simulink model "jumeau_banc_rw"  (R2025b)
settings: Solver=ode23t  StartTime=0.0  StopTime=20  MaxStep=1e-3  RelTol=1e-4
PostLoadFcn:
  | d = fileparts(get_param('jumeau_banc_rw', 'FileName')); addpath(fullfile(d, 'geometrie'), fullfile(d, 'liaison'), fullfile(d, 'pilotage')); clear d
StartFcn:
  | % Jumeau Webots : au lancement, MATLAB envoie les paramètres du Model Workspace à Webots, qui remet le banc en
  | % position de départ, puis ouvre la liaison de télémétrie et la liaison de commande (liaison/pont_banc.m).
  | if strcmp(get_param('jumeau_banc_rw/Procédé', 'LabelModeActiveChoice'), 'Webots')
  |     pont_banc('ouvrir', getVariable(get_param('jumeau_banc_rw', 'ModelWorkspace'), 'config_jumeau'));
  | end
  | pilotage_banc('depart');   % interface de pilotage : nouveau lancement
StopFcn:
  | pont_banc('fermer');
  | pilotage_banc('fin');
model workspace (MATLAB code in the model file):
  | %% Jumeau numérique du banc de stabilisation à 4 roues de réaction (version 3) : paramètres
  | % Ce code est enregistré dans le modèle (Model Explorer > jumeau_banc_rw > Model Workspace).
  | % Origine : (CAO) CAO du banc version 3, (M) mesuré sur le matériel, (F) fiche technique, (Fw) firmware,
  | % (H) hypothèse à mesurer sur le banc. Masses et inerties des pièces : dans chaque bloc de pièce.
  | 
  | %% Montage de l'essai
  | pivot_mm = 25;              % position du pivot de tangage sur le corps : 25, 24, 16, 8, 0, -8 mm (25 : banc équilibré, rangée +24 et paliers remontés de 1 mm)
  | blocage_roulis = 0;         % goupille de blocage : 1 = axe bloqué à 0°, 0 = axe libre
  | blocage_tangage = 0;
  | angle0_roulis_deg = 2;      % position de départ (mise à 0 si l'axe est bloqué)
  | angle0_tangage_deg = -1;
  | g = 9.81;                   % m/s²
  | 
  | %% Pupitre : pilotage manuel des 4 ESC
  | essai_t = 1;                % s, instant de l'échelon d'essai ajouté aux curseurs
  | essai_echelon_us = [0 0 0 0];   % µs, échelon d'essai sur chaque ESC (0 : aucun)
  | 
  | %% Alimentation des ESC
  | V_alim = 12;                % V, alimentation de labo (H : tension réglée)
  | 
  | %% ESC Brushless 30A bidirectionnels (x4)
  | f_trame_esc = 50;           % Hz, une impulsion toutes les 20 ms (Fw : LEDC 50 Hz)
  | imp_neutre = 1500;          % µs, neutre (testé sur le banc)
  | imp_min = 1000;             % µs (Fw)
  | imp_max = 2000;             % µs (Fw)
  | zone_morte_us = 0;          % µs autour du neutre (H)
  | tau_esc = 2e-3;             % s, temps de réponse de l'ESC (H)
  | armement_actif = 1;         % 1 : l'ESC ne pilote le moteur qu'après t_armement au neutre
  | t_armement = 1;             % s (H)
  | fenetre_armement_us = 25;   % µs, écart au neutre accepté pendant l'armement (H)
  | sens_moteurs = [1 1 1 1];   % +1 : au-dessus du neutre, la roue tourne dans le sens +axe (vers l'extérieur) (H : ordre des phases)
  | 
  | %% Moteurs A2212 1400 KV (x4), modèle équivalent continu
  | KV = 1400;                  % tr/min/V (F)
  | Ke = 60/(2*pi*KV);          % V.s/rad
  | Kt = Ke;                    % N.m/A
  | R_moteur = 0.08;            % ohm (H)
  | L_moteur = 30e-6;           % H (H)
  | f_roue = 5e-6;              % N.m.s/rad, frottement visqueux des roulements du moteur (H)
  | 
  | %% Cardan
  | butee_deg = 20;             % débattement de chaque axe (CAO)
  | k_butee = 20;               % N.m/rad, contact goupille-lumière (H)
  | c_butee = 0.2;              % N.m.s/rad (H)
  | b_cardan = 1e-4;            % N.m.s/rad, frottement des roulements 625 (H)
  | k_cables = 0;               % N.m/rad, raideur des deux câbles vers la table (H)
  | 
  | %% BNO055 (mode fusion)
  | T_bno = 0.01;               % s, données de fusion à 100 Hz (F)
  | bruit_bno = 1;              % 1 : bruit de mesure, 0 : capteur parfait
  | sigma_angle_deg = 0.05;     % ° (H)
  | sigma_gyro_dps = 0.1;       % °/s (H)
  | sigma_acc = 0.02;           % m/s² (H)
  | R_montage_bno = eye(3);     % axes du capteur dans le repère du dispositif : eye(3) = remappage AXIS_MAP réglé
  |                             % (la carte est tournée de 90° dans la CAO)
  | 
  | %% Capteurs de vitesse TCRT5000 (x4) : un front à chaque rayon du disque
  | n_rayons = 4;               % rayons du disque vus par tour (CAO : disque d'origine)
  | T_tcrt = 1e-3;              % s, pas de calcul du capteur (les fronts sont datés par interpolation, comme un chronomètre en µs)
  | t_arret_tcrt = 0.2;         % s sans front : la vitesse mesurée retombe à 0 (Fw, à fixer)
  | 
  | %% Pont vers le jumeau Webots (et, plus tard, vers l'ESP32 du banc réel)
  | T_pont = 0.01;              % s, une trame de commande et une trame de télémétrie toutes les 10 ms
  | 
  | %% Essai : maintien au départ et perturbation
  | t_lacher = 2;                % s, le dispositif est tenu à la main à sa position de départ jusqu'à cet instant (0 : libre dès le départ)
  | k_main = 5;                  % N.m/rad, raideur de la main qui tient le dispositif
  | c_main = 0.3;                % N.m.s/rad, son amortissement
  | perturbation_t = 7;          % s, instant de la poussée d'essai
  | perturbation_duree = 0.2;    % s
  | perturbation_couple = [0.02 0.02];   % N.m, couple de la poussée sur [roulis tangage], programmée (0 : aucune ; l'interface de pilotage en ajoute)
  | 
  | %% Grandeurs dérivées
  | assert(any(pivot_mm == [25 24 16 8 0 -8]), 'pivot_mm : 25, 24, 16, 8, 0, -8');
  | q0_deg = [angle0_roulis_deg angle0_tangage_deg] .* ([blocage_roulis blocage_tangage] == 0);
  | config_jumeau = [pivot_mm; blocage_roulis; blocage_tangage; q0_deg(:); V_alim; f_trame_esc; imp_neutre; imp_min; imp_max; ...
  |     zone_morte_us; tau_esc; armement_actif; t_armement; fenetre_armement_us; sens_moteurs(:); Ke; Kt; R_moteur; L_moteur; ...
  |     f_roue; butee_deg; k_butee; c_butee; b_cardan; k_cables; g; T_bno; bruit_bno; sigma_angle_deg; sigma_gyro_dps; ...
  |     sigma_acc; n_rayons; t_arret_tcrt; T_tcrt; R_montage_bno(:); T_pont; t_lacher; k_main; c_main];   % 51 valeurs envoyées au jumeau Webots au lancement
  | 
  | %% Commande bas niveau : une boucle de vitesse par roue, avec observateur CFO (méthode du TP2, ramenée à la vitesse)
  | J_roue = 1.562e-4;          % kg.m², inertie d'une roue autour de son axe : disque, vis, cloche du moteur (CAO)
  | T_cbn = 1/f_trame_esc;      % s, période de calcul de la commande : celle des ESC, qui ne lisent qu'une impulsion toutes les 20 ms
  | wc_roue = [10 10 10 10];    % rad/s, rapidité du suivi de vitesse de chaque roue (pôle de l'erreur en -wc)
  | wo_roue = [5 5 5 5];        % rad/s, rapidité du CFO de chaque roue (pôles en -wo et -4 wo) ; au-delà de 10, il devient instable à 20 ms
  | imp_cmd_min = 1375;         % µs, limites des impulsions commandées : vitesse conseillée des disques, 3 900 tr/min
  | imp_cmd_max = 1625;         % µs
  | w_aveugle = 45;             % rad/s, en dessous (vitesse du modèle), le TCRT5000 voit mal la roue : le CFO ne se corrige plus sur la mesure
  | 
  | %% Consigne d'essai des roues : ajoutée à la consigne qui vient de la conversion (0 tant qu'elle est vide)
  | essai_roue_t1 = 2;                  % s, départ vers le premier palier
  | essai_roue_vitesse1 = [0 0 0 0];  % rad/s, premier palier de chaque roue (0 : la roue reste à l'arrêt)
  | essai_roue_t2 = 6;                  % s, départ vers le second palier
  | essai_roue_vitesse2 = [0 0 0 0];    % rad/s, second palier de chaque roue
  | essai_roue_acc = 300;               % rad/s², pente des rampes entre les paliers
  | 
  | %% Commande bas niveau : grandeurs calculées
  | % modèle local d'une roue : d(omega)/dt = -a1 omega + a0 V + d
  | a0_roue = Kt/(R_moteur*J_roue) * [1 1 1 1];                % rad/s² par volt
  | a1_roue = (Kt*Ke/R_moteur + f_roue)/J_roue * [1 1 1 1];    % 1/s
  | K_roue = wc_roue - a1_roue;                                % retour d'état : erreur en -(a1 + K) = -wc
  | l1_roue = 5*wo_roue;                                       % CFO
  | lambda_roue = 4/5*wo_roue;
  | 
  | %% Référence : angles demandés au dispositif, en polynômes de degré 5 entre deux paliers
  | ref_t = [2 12];              % s, instant de départ vers chaque palier
  | ref_roulis_deg = [0 5];      % °, roulis demandé à chaque palier
  | ref_tangage_deg = [0 0];     % °, tangage demandé à chaque palier
  | ref_duree = 1.5;             % s, durée du passage d'un palier au suivant
  | 
  | %% Commande haut niveau : une boucle par axe [roulis tangage], placement de pôles basé sur l'observateur CFO (TP2)
  | T_chn = T_cbn;               % s, période de calcul : celle de la commande bas niveau et des ESC
  | t_depart = t_lacher;         % s, mise en marche de la commande : au moment où la main lâche le dispositif
  | wc_axe = [4 4];              % rad/s, rapidité du suivi d'angle de chaque axe
  | xi_axe = [1 1];              % amortissement
  | wo_axe = [3 3];              % rad/s, rapidité du CFO de chaque axe (pôles en -wo et -4 wo, double) ; au-delà de 4, le couple s'agite
  | desat_active = 0;            % 1 : la référence est décalée pour ramener les roues vers leur vitesse de repos
  | T_desat = 5;                 % s, constante de temps de ce retour
  | desat_max_deg = 15;          % °, décalage maximal de la référence
  | 
  | %% Conversion : couples des deux axes vers les 4 roues
  | w_repos = 200;               % rad/s, vitesse de repos des 4 roues : elles tournent toujours, le TCRT5000 les voit toujours
  | t_roues = t_armement + 0.2;  % s, mise en rotation des roues, une fois les ESC armés
  | acc_roue_max = 300;          % rad/s², accélération maximale demandée à une roue
  | w_roue_min = 60;             % rad/s, vitesses limites demandées à une roue
  | w_roue_max = 400;            % rad/s (disques : 3 900 tr/min conseillés, soit 408 rad/s)
  | 
  | %% Masses et inerties utilisées par la commande (CAO du banc version 3)
  | m_disp = 1.2615;             % kg, dispositif et ses 4 roues
  | zG_disp = 24.977e-3;         % m, hauteur de son centre de masse sur le corps (le pivot est à pivot_mm)
  | Ixx_disp_24 = 8.2684e-3;     % kg.m², inertie du dispositif autour du roulis, pivot à +24 mm
  | Iyy_disp_24 = 8.2786e-3;     % kg.m², autour du tangage, pivot à +24 mm
  | m_croix = 0.0755;            % kg, croisillon et paliers (ne tournent qu'en roulis)
  | zG_croix = 0.257e-3;         % m, hauteur de leur centre de masse au-dessus de l'axe de roulis
  | Ixx_croix = 2.073e-4;        % kg.m²
  | 
  | %% Commande haut niveau et conversion : grandeurs calculées
  | % modèle local d'un axe : d²(theta)/dt² = -a1 d(theta)/dt + a0 C + d, avec C le couple demandé aux roues
  | hz = zG_disp - pivot_mm/1000;                                    % m, centre de masse du dispositif au-dessus du pivot
  | I_axe = [Ixx_disp_24 + Ixx_croix, Iyy_disp_24] + m_disp*(hz^2 - (zG_disp - 0.024)^2) - 2*J_roue;   % kg.m²
  | mgh_axe = g*[m_disp*hz + m_croix*zG_croix, m_disp*hz];           % N.m/rad, couple de pesanteur par radian d'inclinaison
  | a0_axe = 1./I_axe;                                               % rad/s² par N.m
  | a1_axe = b_cardan./I_axe;                                        % 1/s
  | k1_axe = wc_axe.^2;                                              % retour d'état : s² + 2 xi wc s + wc²
  | k2_axe = 2*xi_axe.*wc_axe - a1_axe;
  | l1_axe = 9*wo_axe;                                               % CFO du TP2
  | l2_axe = 12*wo_axe.^2;
  | lambda_axe = 4/3*wo_axe;
  | C_max = 2*J_roue*cosd(45)*acc_roue_max;                          % N.m, couple maximal demandé sur un axe
  | k_desat = desat_active.*sign(mgh_axe + (mgh_axe == 0))./(max(abs(mgh_axe), 1e-3)*T_desat);            % rad par N.m.s
  | sx_roues = [1 -1 -1 1];                                          % signe de cos(45°, 135°, 225°, 315°) : part de chaque roue sur le roulis
  | sy_roues = [1 1 -1 -1];                                          % signe de sin : part sur le tangage
  | M_conv = -[sx_roues(:) sy_roues(:)]/(4*J_roue*cosd(45));         % accélération des 4 roues pour un couple [roulis; tangage]
  | 
  | %% Perception : des mesures à l'état du banc
  | T_perception = T_bno;        % s, période de calcul : celle du BNO055
  | tau_desequilibre = 2;        % s, constante de temps du filtre du couple extérieur et du déséquilibre
  | 
  | %% Pilotage par l'interface (pilotage/pilote_banc.m)
  | manche_max_deg = 15;         % °, limite de sécurité de l'inclinaison demandée par le manche (l'interface règle l'amplitude)
  | w_manche = 3;                % rad/s, rapidité avec laquelle la référence rejoint le manche (second ordre critique)
  | T_affichage = 0.1;           % s, rafraîchissement de l'interface
undefined symbols (not defined in the file): DiscIntNeverNeededParam, X, Y, Z
libraries: sm_lib x256, nesl_utility x24, simulink x7
(part 2 of 8)

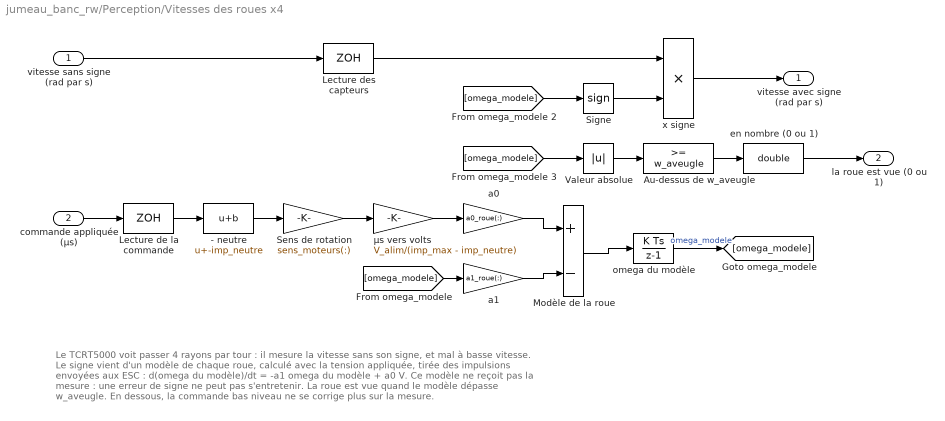
== system jumeau_banc_rw/Perception/Vitesses des roues x4 ==
  note: Le TCRT5000 voit passer 4 rayons par tour : il mesure la vitesse sans son signe, et mal à basse vitesse.
      | Le signe vient d'un modèle de chaque roue, calculé avec la tension appliquée, tirée des impulsions envoyées aux ESC :
      | d(omega du modèle)/dt = -a1 omega du modèle + a0 V. Ce modèle ne reçoit pas la mesure : une erreur de signe ne peut pas s'entretenir.
      | La roue est vue quand le modèle dépasse w_aveugle. En dessous, la commande bas niveau ne se corrige plus sur la mesure.
  vitesse sans signe (rad par s) : Inport
  commande appliquée (µs) : Inport  Port=2
  - neutre : Bias  Bias=-imp_neutre  SaturateOnIntegerOverflow=off
  Au-dessus de w_aveugle : simulink/Logic and Bit Operations/Compare To Constant  relop=>=  const=w_aveugle  OutDataTypeStr=boolean
  Lecture de la commande : ZeroOrderHold  SampleTime=T_perception
  Lecture des capteurs : ZeroOrderHold  SampleTime=T_perception
  Modèle de la roue : Sum  Inputs=+-
  Sens de rotation : Gain  Gain=sens_moteurs(:)
  Signe : Signum
  Valeur absolue : Abs  SaturateOnIntegerOverflow=off
  a0 : Gain  Gain=a0_roue(:)
  a1 : Gain  Gain=a1_roue(:)
  en nombre (0 ou 1) : DataTypeConversion  OutDataTypeStr=double  SaturateOnIntegerOverflow=off  RndMeth=Floor
  omega du modèle : DiscreteIntegrator  gainval=1  SampleTime=T_perception  ICPrevOutput=DiscIntNeverNeededParam  ICPrevScaledInput=DiscIntNeverNeededParam
  x signe : Product
  µs vers volts : Gain  Gain=V_alim/(imp_max - imp_neutre)
  vitesse avec signe (rad par s) : Outport
  la roue est vue (0 ou 1) : Outport  Port=2
  wires:
  vitesse sans signe (rad par s)/1 -> Lecture des capteurs/1
  Lecture des capteurs/1 -> x signe/1
  commande appliquée (µs)/1 -> Lecture de la commande/1
  Lecture de la commande/1 -> - neutre/1
  - neutre/1 -> Sens de rotation/1
  Sens de rotation/1 -> µs vers volts/1
  µs vers volts/1 -> a0/1
  a0/1 -> Modèle de la roue/1
  [omega_modele] -> a1/1
  a1/1 -> Modèle de la roue/2
  Modèle de la roue/1 -> omega du modèle/1
  omega du modèle/1 -> [omega_modele]  "omega_modele"
  [omega_modele] -> Signe/1
  Signe/1 -> x signe/2
  x signe/1 -> vitesse avec signe (rad par s)/1
  [omega_modele] -> Valeur absolue/1
  Valeur absolue/1 -> Au-dessus de w_aveugle/1
  Au-dessus de w_aveugle/1 -> en nombre (0 ou 1)/1
  en nombre (0 ou 1)/1 -> la roue est vue (0 ou 1)/1

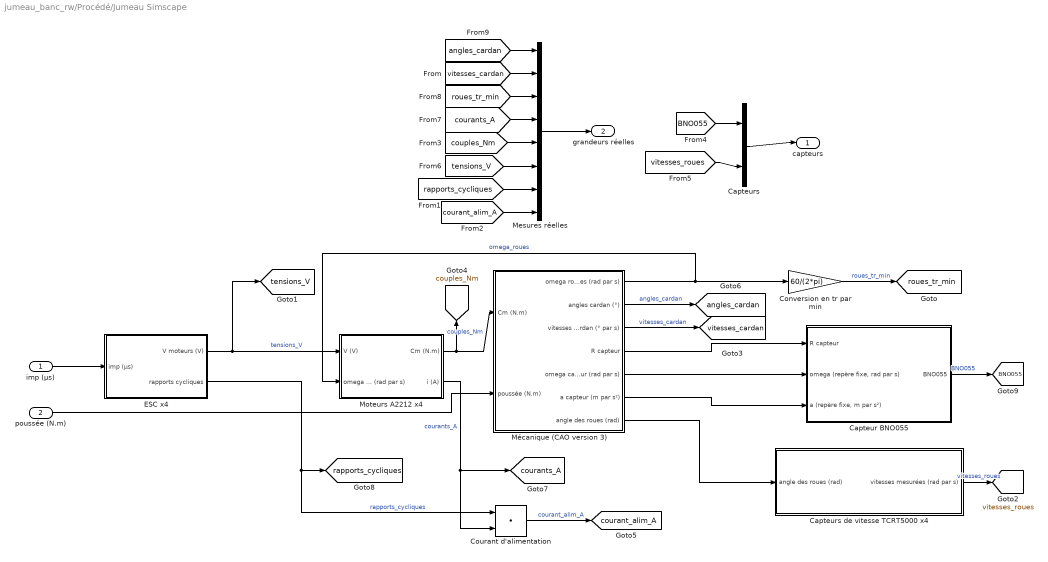
== system jumeau_banc_rw/Procédé/Jumeau Simscape ==
  imp (µs) : Inport
  poussée (N.m) : Inport  Port=2
  Capteur BNO055 : Subsystem
  Capteurs : BusCreator  Inputs=2
  Capteurs de vitesse TCRT5000 x4 : Subsystem
  Conversion en tr par min : Gain  Gain=60/(2*pi)
  Courant d'alimentation : DotProduct  OutDataTypeStr=Inherit: Inherit via internal rule
  ESC x4 : Subsystem
  Mesures réelles : BusCreator  Description=Grandeurs du banc réel, sans bruit : ce que le BNO055 et l'ESP32 ne voient pas.  Inputs=8
  Moteurs A2212 x4 : Subsystem
  Mécanique (CAO version 3) : Subsystem
  capteurs : Outport
  grandeurs réelles : Outport  Port=2
  tag scope: BNO055=global, angles_cardan=global, couples_Nm=global, courant_alim_A=global, courants_A=global, rapports_cycliques=global, roues_tr_min=global, tensions_V=global, vitesses_cardan=global, vitesses_roues=global
  wires:
  imp (µs)/1 -> ESC x4/1(imp (µs))
  ESC x4/1(V moteurs (V)) -> [tensions_V], Moteurs A2212 x4/1(V (V))  "tensions_V"
  Moteurs A2212 x4/1(Cm (N.m)) -> Mécanique (CAO version 3)/1(Cm (N.m)), [couples_Nm]  "couples_Nm"
  Mécanique (CAO version 3)/1(omega roues (rad par s)) -> Conversion en tr par min/1, Moteurs A2212 x4/2(omega roues (rad par s))  "omega_roues"
  Mécanique (CAO version 3)/4(R capteur) -> Capteur BNO055/1(R capteur)
  Mécanique (CAO version 3)/5(omega capteur (rad par s)) -> Capteur BNO055/2("omega (repère fixe, rad par s)")
  Mécanique (CAO version 3)/6(a capteur (m par s²)) -> Capteur BNO055/3("a (repère fixe, m par s²)")
  Mécanique (CAO version 3)/7(angle des roues (rad)) -> Capteurs de vitesse TCRT5000 x4/1(angle des roues (rad))
  Capteurs/1 -> capteurs/1
  ESC x4/2(rapports cycliques) -> [rapports_cycliques], Courant d'alimentation/1  "rapports_cycliques"
  Moteurs A2212 x4/2(i (A)) -> Courant d'alimentation/2, [courants_A]  "courants_A"
  Mécanique (CAO version 3)/2(angles cardan (°)) -> [angles_cardan]  "angles_cardan"
  Mécanique (CAO version 3)/3(vitesses cardan (° par s)) -> [vitesses_cardan]  "vitesses_cardan"
  Mesures réelles/1 -> grandeurs réelles/1
  [angles_cardan] -> Mesures réelles/1
  [vitesses_cardan] -> Mesures réelles/2
  Conversion en tr par min/1 -> [roues_tr_min]  "roues_tr_min"
  [roues_tr_min] -> Mesures réelles/3
  [courants_A] -> Mesures réelles/4
  [couples_Nm] -> Mesures réelles/5
  [tensions_V] -> Mesures réelles/6
  [rapports_cycliques] -> Mesures réelles/7
  [courant_alim_A] -> Mesures réelles/8
  Courant d'alimentation/1 -> [courant_alim_A]  "courant_alim_A"
  [BNO055] -> Capteurs/1
  [vitesses_roues] -> Capteurs/2
  Capteur BNO055/1(BNO055) -> [BNO055]  "BNO055"
  Capteurs de vitesse TCRT5000 x4/1(vitesses mesurées (rad par s)) -> [vitesses_roues]  "vitesses_roues"
  poussée (N.m)/1 -> Mécanique (CAO version 3)/2(poussée (N.m))

== system jumeau_banc_rw/Procédé/Jumeau Webots ==
  note: Jumeau Webots : le même banc, calculé par Webots (physique ODE, vue 3D). Lancer Webots avant la simulation :
      | ouvrir webots/worlds/banc_stabilisation.wbt, puis lancer ce modèle. Webots avance au rythme de Simulink, 10 ms par trame.
      | Liaison locale (liaison/pont_banc.m) : télémétrie reçue sur le port 5005, commande envoyée sur le port 5006 ; ce sont les trames
      | du banc réel : il suffira de remplacer Webots par l'ESP32.
      | Au lancement, les paramètres du Model Workspace (ESC, moteurs, cardan, capteurs, montage de l'essai) sont envoyés à Webots
      | (port 5007, rappel StartFcn du modèle) : MATLAB reste la seule source des réglages. Webots remet alors le banc en position de départ.
  note: Trame de commande du jumeau : les 13 octets de l'ESP32, plus la poussée d'essai (8 octets) avant la somme de contrôle, soit 21 octets.
  imp (µs) : Inport
  poussée (N.m) : Inport  Port=2
  Capteurs : BusCreator  Inputs=2
  Décodage de la télémétrie : MATLAB Function  TreatAsAtomicUnit=on
  Envoi au procédé : MATLAB Function  TreatAsAtomicUnit=on
  Mesures réelles : BusCreator  Inputs=8
  Poussée toutes les T_pont : ZeroOrderHold  SampleTime=T_pont
  Registres : BusCreator  Description=Ce que lit l'ESP32 par I2C : euler = [cap roulis tangage] (°), gyro (°/s), quat, acc (m/s²).  Inputs=4
  Réception du procédé : MATLAB Function  TreatAsAtomicUnit=on
  Trame de commande : MATLAB Function  TreatAsAtomicUnit=on
  Trame valide (1) : Display
  Une trame toutes les T_pont : ZeroOrderHold  SampleTime=T_pont
  capteurs : Outport
  grandeurs réelles : Outport  Port=2
  wires:
  imp (µs)/1 -> Une trame toutes les T_pont/1
  Une trame toutes les T_pont/1 -> Trame de commande/1(imp)
  Trame de commande/1(trame) -> Envoi au procédé/1(trame)
  Réception du procédé/1(trame) -> Décodage de la télémétrie/1(trame)
  Décodage de la télémétrie/1(euler) -> Registres/1  "euler"
  Décodage de la télémétrie/2(gyro) -> Registres/2  "gyro"
  Décodage de la télémétrie/3(quat) -> Registres/3  "quat"
  Décodage de la télémétrie/4(acc) -> Registres/4  "acc"
  Registres/1 -> Capteurs/1  "BNO055"
  Décodage de la télémétrie/5(w_mes) -> Capteurs/2  "vitesses_roues"
  Capteurs/1 -> capteurs/1
  Décodage de la télémétrie/6(angles) -> Mesures réelles/1  "angles_cardan"
  Décodage de la télémétrie/7(vitesses) -> Mesures réelles/2  "vitesses_cardan"
  Décodage de la télémétrie/8(tr_min) -> Mesures réelles/3  "roues_tr_min"
  Décodage de la télémétrie/9(courants) -> Mesures réelles/4  "courants_A"
  Décodage de la télémétrie/10(couples) -> Mesures réelles/5  "couples_Nm"
  Décodage de la télémétrie/11(tensions) -> Mesures réelles/6  "tensions_V"
  Décodage de la télémétrie/12(rapports) -> Mesures réelles/7  "rapports_cycliques"
  Décodage de la télémétrie/13(i_alim) -> Mesures réelles/8  "courant_alim_A"
  Mesures réelles/1 -> grandeurs réelles/1
  Décodage de la télémétrie/14(ok) -> Trame valide (1)/1
  poussée (N.m)/1 -> Poussée toutes les T_pont/1
  Poussée toutes les T_pont/1 -> Trame de commande/2(poussee)

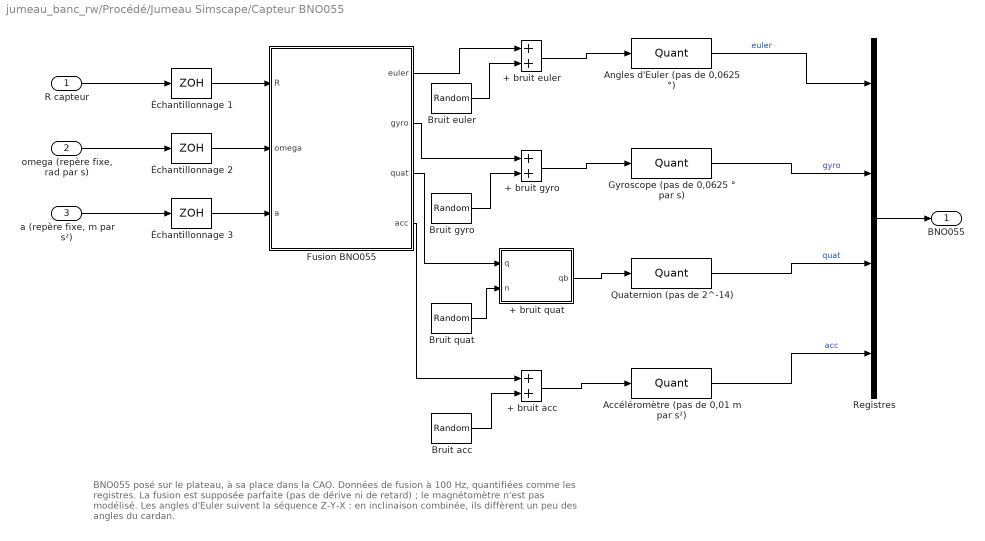
== system jumeau_banc_rw/Procédé/Jumeau Simscape/Capteur BNO055 ==
  note: BNO055 posé sur le plateau, à sa place dans la CAO. Données de fusion à 100 Hz, quantifiées comme les registres.
      | La fusion est supposée parfaite (pas de dérive ni de retard) ; le magnétomètre n'est pas modélisé.
      | Les angles d'Euler suivent la séquence Z-Y-X : en inclinaison combinée, ils diffèrent un peu des angles du cardan.
  R capteur : Inport
  "omega (repère fixe, rad par s)" : Inport  Port=2
  "a (repère fixe, m par s²)" : Inport  Port=3
  + bruit acc : Sum
  + bruit euler : Sum
  + bruit gyro : Sum
  + bruit quat : MATLAB Function  TreatAsAtomicUnit=on
  Accéléromètre (pas de 0,01 m par s²) : Quantizer  QuantizationInterval=0.01
  Angles d'Euler (pas de 0,0625 °) : Quantizer  QuantizationInterval=1/16
  Bruit acc : RandomNumber  Mean=[0; 0; 0]  Variance=(bruit_bno * sigma_acc)^2  Seed=[41 42 43]  SampleTime=T_bno
  Bruit euler : RandomNumber  Mean=[0; 0; 0]  Variance=(bruit_bno * sigma_angle_deg)^2  Seed=[11 12 13]  SampleTime=T_bno
  Bruit gyro : RandomNumber  Mean=[0; 0; 0]  Variance=(bruit_bno * sigma_gyro_dps)^2  Seed=[21 22 23]  SampleTime=T_bno
  Bruit quat : RandomNumber  Mean=[0; 0; 0]  Variance=(bruit_bno * sigma_angle_deg * pi/180)^2  Seed=[41 42 43]  SampleTime=T_bno
  Fusion BNO055 : MATLAB Function  TreatAsAtomicUnit=on
  Gyroscope (pas de 0,0625 ° par s) : Quantizer  QuantizationInterval=1/16
  Quaternion (pas de 2^-14) : Quantizer  QuantizationInterval=1/2^14
  Registres : BusCreator  Description=Ce que lit l'ESP32 par I2C : euler = [cap roulis tangage] (°), gyro (°/s), quat, acc (m/s²).  Inputs=4
  Échantillonnage 1 : ZeroOrderHold  SampleTime=T_bno
  Échantillonnage 2 : ZeroOrderHold  SampleTime=T_bno
  Échantillonnage 3 : ZeroOrderHold  SampleTime=T_bno
  BNO055 : Outport
  wires:
  R capteur/1 -> Échantillonnage 1/1
  "omega (repère fixe, rad par s)"/1 -> Échantillonnage 2/1
  "a (repère fixe, m par s²)"/1 -> Échantillonnage 3/1
  Échantillonnage 1/1 -> Fusion BNO055/1(R)
  Échantillonnage 2/1 -> Fusion BNO055/2(omega)
  Échantillonnage 3/1 -> Fusion BNO055/3(a)
  Fusion BNO055/1(euler) -> + bruit euler/1
  Bruit euler/1 -> + bruit euler/2
  + bruit euler/1 -> Angles d'Euler (pas de 0,0625 °)/1
  Fusion BNO055/2(gyro) -> + bruit gyro/1
  Bruit gyro/1 -> + bruit gyro/2
  + bruit gyro/1 -> Gyroscope (pas de 0,0625 ° par s)/1
  Fusion BNO055/4(acc) -> + bruit acc/1
  Bruit acc/1 -> + bruit acc/2
  + bruit acc/1 -> Accéléromètre (pas de 0,01 m par s²)/1
  Angles d'Euler (pas de 0,0625 °)/1 -> Registres/1  "euler"
  Gyroscope (pas de 0,0625 ° par s)/1 -> Registres/2  "gyro"
  Quaternion (pas de 2^-14)/1 -> Registres/3  "quat"
  Accéléromètre (pas de 0,01 m par s²)/1 -> Registres/4  "acc"
  Registres/1 -> BNO055/1
  Fusion BNO055/3(quat) -> + bruit quat/1(q)
  Bruit quat/1 -> + bruit quat/2(n)
  + bruit quat/1(qb) -> Quaternion (pas de 2^-14)/1

== system jumeau_banc_rw/Procédé/Jumeau Simscape/Capteurs de vitesse TCRT5000 x4 ==
  note: TCRT5000 : un capteur par roue, sur sa potence, devant la face extérieure du disque. Il voit passer les 4 rayons.
      | Vitesse = (2 pi / 4) / durée entre deux fronts, sans signe ; retour à 0 après t_arret_tcrt sans front.
      | La valeur est lue toutes les T_pont (10 ms), comme dans la trame de télémétrie de l'ESP32.
  angle des roues (rad) : Inport
  Lecture à chaque trame : ZeroOrderHold  SampleTime=T_pont
  Mesure de la période : MATLAB Function  TreatAsAtomicUnit=on
  Pas du capteur : ZeroOrderHold  SampleTime=T_tcrt
  vitesses mesurées (rad par s) : Outport
  wires:
  angle des roues (rad)/1 -> Pas du capteur/1
  Pas du capteur/1 -> Mesure de la période/1(theta)
  Mesure de la période/1(w) -> Lecture à chaque trame/1
  Lecture à chaque trame/1 -> vitesses mesurées (rad par s)/1

== system jumeau_banc_rw/Procédé/Jumeau Simscape/ESC x4 ==
  note: ESC : à chaque trame (20 ms), l'impulsion fixe le rapport cyclique u = (imp - 1500)/500,
      | puis la tension moyenne appliquée au moteur V = u V_alim, avec le temps de réponse tau_esc.
      | Le courant pris à l'alimentation vaut la somme des u i (rapports cycliques x courants moteurs).
  imp (µs) : Inport
  Armement : MATLAB Function  TreatAsAtomicUnit=on
  Inverse de tau_esc : Gain  Gain=1/tau_esc
  Lecture des trames (50 Hz) : ZeroOrderHold  SampleTime=1/f_trame_esc
  Plage 1000-2000 µs : Saturate  UpperLimit=imp_max  LowerLimit=imp_min
  Rapport cyclique : Gain  Gain=1/(imp_max - imp_neutre)
  Sens de rotation : Gain  Gain=sens_moteurs(:)
  Tension moyenne : Integrator  InitialCondition=[0; 0; 0; 0]
  Zone morte : DeadZone  LowerValue=-zone_morte_us  UpperValue=zone_morte_us
  e : Sum  Inputs=+-
  x V_alim : Gain  Gain=V_alim
  x armé : Product
  Écart au neutre : Bias  Bias=-imp_neutre  SaturateOnIntegerOverflow=off
  V moteurs (V) : Outport
  rapports cycliques : Outport  Port=2
  wires:
  imp (µs)/1 -> Lecture des trames (50 Hz)/1
  Lecture des trames (50 Hz)/1 -> Plage 1000-2000 µs/1, Armement/1(imp)
  Plage 1000-2000 µs/1 -> Écart au neutre/1
  Écart au neutre/1 -> Zone morte/1
  Zone morte/1 -> Rapport cyclique/1
  Rapport cyclique/1 -> x armé/1
  Armement/1(arme) -> x armé/2
  x armé/1 -> Sens de rotation/1
  Sens de rotation/1 -> x V_alim/1, rapports cycliques/1
  x V_alim/1 -> e/1
  e/1 -> Inverse de tau_esc/1
  Inverse de tau_esc/1 -> Tension moyenne/1
  Tension moyenne/1 -> V moteurs (V)/1, e/2

== system jumeau_banc_rw/Procédé/Jumeau Simscape/Moteurs A2212 x4 ==
  note: A2212, modèle équivalent continu (comme le TP1), pour chacun des 4 moteurs :
      | L di/dt = V - R i - Ke omega,   Cm = Kt i.
      | omega est la vitesse de la roue par rapport au dispositif ; Cm agit sur la roue et, en réaction, sur le dispositif.
      | Le frottement des roulements (f_roue) et l'inertie (CAO) sont dans la mécanique.
  V (V) : Inport
  omega roues (rad par s) : Inport  Port=2
  Courant i : Integrator  InitialCondition=[0; 0; 0; 0]
  Inverse de L : Gain  Gain=1/L_moteur
  Ke (f.c.é.m.) : Gain  Gain=Ke
  Kt : Gain  Gain=Kt
  R : Gain  Gain=R_moteur
  Somme des tensions : Sum  Inputs=+--
  Cm (N.m) : Outport
  i (A) : Outport  Port=2
  wires:
  V (V)/1 -> Somme des tensions/1
  Somme des tensions/1 -> Inverse de L/1
  Inverse de L/1 -> Courant i/1
  Courant i/1 -> R/1, i (A)/1, Kt/1
  Kt/1 -> Cm (N.m)/1
  R/1 -> Somme des tensions/2
  omega roues (rad par s)/1 -> Ke (f.c.é.m.)/1
  Ke (f.c.é.m.)/1 -> Somme des tensions/3

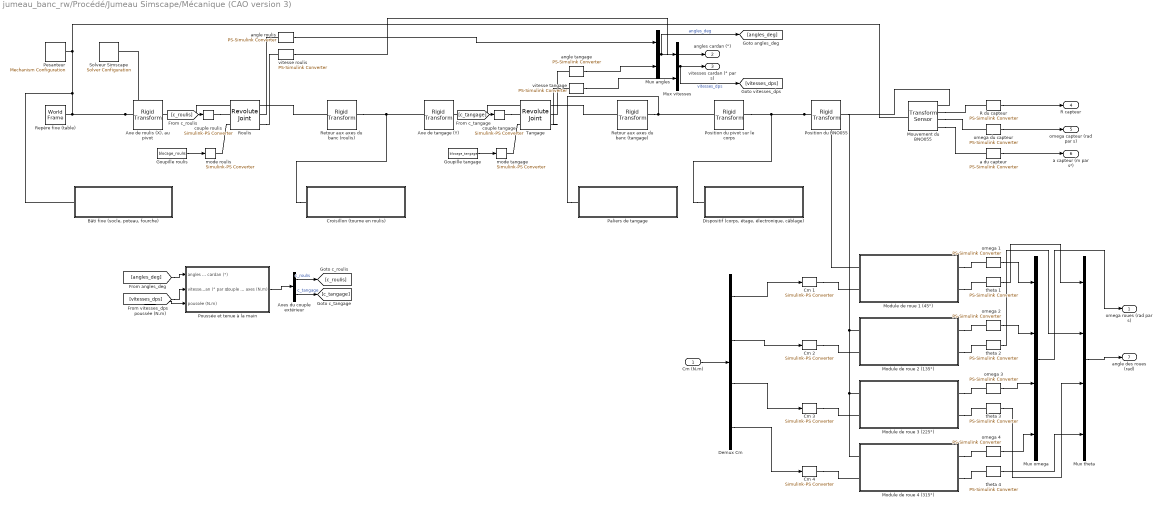
== system jumeau_banc_rw/Procédé/Jumeau Simscape/Mécanique (CAO version 3) ==
  Cm (N.m) : Inport
  poussée (N.m) : Inport  Port=2
  "Axe de roulis (X), au pivot" : sm_lib/Frames and Transforms/Rigid Transform  Description=Le centre de rotation (centre du croisillon) est fixe, à 24 mm au-dessus de l'origine du repère fixe.  RotationMethod=StandardAxis  FollAlignAxisA=+X  BaseAlignAxisA=+Y  FollAlignAxisB=+Y  BaseAlignAxisB=+Z  RotationStandardAxis=+Y  RotationAngle=90  RotationAngleUnits=deg  RotationArbitraryAxis=[0 0 1]  RotationSequenceAxes=FollowerAxes  RotationSequence=XYX  RotationSequenceAngles=[0 0 0]  RotationSequenceAnglesUnits=deg  RotationMatrix=[1 0 0;0 1 0;0 0 1]  Quaternion=[1 0 0 0]  TranslationMethod=Cartesian  TranslationCartesianOffset=[0 0 24]  TranslationCartesianOffsetUnits=mm  TranslationStandardAxis=+Z  TranslationStandardOffset=0  TranslationStandardOffsetUnits=m  TranslationROffset=0  TranslationROffsetUnits=m  TranslationThetaOffset=0  TranslationThetaOffsetUnits=deg  TranslationZOffset=0  TranslationZOffsetUnits=m
  Axe de tangage (Y) : sm_lib/Frames and Transforms/Rigid Transform  RotationMethod=StandardAxis  FollAlignAxisA=+X  BaseAlignAxisA=+Y  FollAlignAxisB=+Y  BaseAlignAxisB=+Z  RotationStandardAxis=+X  RotationAngle=-90  RotationAngleUnits=deg  RotationArbitraryAxis=[0 0 1]  RotationSequenceAxes=FollowerAxes  RotationSequence=XYX  RotationSequenceAngles=[0 0 0]  RotationSequenceAnglesUnits=deg  RotationMatrix=[1 0 0;0 1 0;0 0 1]  Quaternion=[1 0 0 0]  TranslationMethod=None  TranslationCartesianOffset=[0 0 0]  TranslationCartesianOffsetUnits=m  TranslationStandardAxis=+Z  TranslationStandardOffset=0  TranslationStandardOffsetUnits=m  TranslationROffset=0  TranslationROffsetUnits=m  TranslationThetaOffset=0  TranslationThetaOffsetUnits=deg  TranslationZOffset=0  TranslationZOffsetUnits=m
  Axes du couple extérieur : Demux  Outputs=2
  "Bâti fixe (socle, poteau, fourche)" : Subsystem  Description=repère fixe : origine au centre du corps au repos pour le pivot à 24 mm, Z vers le haut, X roulis, Y tangage
  Cm {1..4} (4 alike) : nesl_utility/Simulink-PS Converter  PhysicalDomain=network_engine_domain  SubClassName=ps_input  LeftPortType=input  RightPortType=output  PseudoPeriodic=off  Frequencies=[]  NoiseDistribution=none  NoiseParameters=[]  Unit=N*m  AffineConversion=off  FilteringAndDerivatives=provide  SimscapeFilterOrder=1  InputFilterTimeConstant=0.001  UdotUserProvided=0
  Croisillon (tourne en roulis) : Subsystem  Description=repère : centre du croisillon (pivot), axes du banc tournés du roulis
  Demux Cm : Demux
  "Dispositif (corps, étage, électronique, câblage)" : Subsystem  Description=repère : origine du dispositif (centre du corps, hauteur des axes des moteurs)
  Goupille roulis : Constant  Value=blocage_roulis
  Goupille tangage : Constant  Value=blocage_tangage
  Module de roue 1 (45°) : Subsystem
  Module de roue 2 (135°) : Subsystem
  Module de roue 3 (225°) : Subsystem
  Module de roue 4 (315°) : Subsystem
  Mouvement du BNO055 : sm_lib/Frames and Transforms/Transform Sensor  MeasurementFrame=World  RotationSequence=XYX  SenseAngle=off  SenseAxis=off  SenseQ=off  SenseR=on  SenseRotationSequence=off  SenseOmegaX=off  SenseOmegaY=off  SenseOmegaZ=off  SenseOmega=on  SenseQDot=off  SenseRDot=off  SenseRotationSequenceDot=off  SenseAlphaX=off  SenseAlphaY=off  SenseAlphaZ=off  SenseAlpha=off  SenseQDDot=off  SenseRDDot=off  SenseX=off  SenseY=off  SenseZ=off  SenseXYZ=off  SenseRad=off  SenseAzim=off  SenseDist=off  SenseInc=off  SenseXDot=off  SenseYDot=off  SenseZDot=off  SenseXYZDot=off  SenseRadDot=off  SenseAzimDot=off  SenseDistDot=off  SenseIncDot=off  SenseXDDot=off  SenseYDDot=off  SenseZDDot=off  SenseXYZDDot=on  SenseRadDDot=off  SenseAzimDDot=off  SenseDistDDot=off  SenseIncDDot=off
  Mux angles : Mux  Inputs=2
  Mux omega : Mux
  Mux theta : Mux
  Mux vitesses : Mux  Inputs=2
  Paliers de tangage : Subsystem  Description=repère : pivot, axes du dispositif
  Pesanteur : sm_lib/Utilities/Mechanism Configuration  UniformGravity=Constant  GravityVector=[0 0 -g]  GravityVectorUnits=m/s^2  LinearizationDelta=0.001  JointModeTransitionNonlinearIterations=2
  Position du BNO055 : sm_lib/Frames and Transforms/Rigid Transform  Description=Centre de la carte GY-BNO055 dans la CAO (RW-32), dans le repère du dispositif.  RotationMethod=None  FollAlignAxisA=+X  BaseAlignAxisA=+Y  FollAlignAxisB=+Y  BaseAlignAxisB=+Z  RotationStandardAxis=+Z  RotationAngle=0  RotationAngleUnits=deg  RotationArbitraryAxis=[0 0 1]  RotationSequenceAxes=FollowerAxes  RotationSequence=XYX  RotationSequenceAngles=[0 0 0]  RotationSequenceAnglesUnits=deg  RotationMatrix=[1 0 0;0 1 0;0 0 1]  Quaternion=[1 0 0 0]  TranslationMethod=Cartesian  TranslationCartesianOffset=[-1.85143 2.14674e-16 65.331]  TranslationCartesianOffsetUnits=mm  TranslationStandardAxis=+Z  TranslationStandardOffset=0  TranslationStandardOffsetUnits=m  TranslationROffset=0  TranslationROffsetUnits=m  TranslationThetaOffset=0  TranslationThetaOffsetUnits=deg  TranslationZOffset=0  TranslationZOffsetUnits=m
  Position du pivot sur le corps : sm_lib/Frames and Transforms/Rigid Transform  Description=Les paliers se vissent sur l'une des 5 paires d'inserts du corps (pivot_mm). Le repère suivant est l'origine du dispositif : centre du corps, à la hauteur des axes des moteurs.  RotationMethod=None  FollAlignAxisA=+X  BaseAlignAxisA=+Y  FollAlignAxisB=+Y  BaseAlignAxisB=+Z  RotationStandardAxis=+Z  RotationAngle=0  RotationAngleUnits=deg  RotationArbitraryAxis=[0 0 1]  RotationSequenceAxes=FollowerAxes  RotationSequence=XYX  RotationSequenceAngles=[0 0 0]  RotationSequenceAnglesUnits=deg  RotationMatrix=[1 0 0;0 1 0;0 0 1]  Quaternion=[1 0 0 0]  TranslationMethod=Cartesian  TranslationCartesianOffset=[0 0 -pivot_mm]  TranslationCartesianOffsetUnits=mm  TranslationStandardAxis=+Z  TranslationStandardOffset=0  TranslationStandardOffsetUnits=m  TranslationROffset=0  TranslationROffsetUnits=m  TranslationThetaOffset=0  TranslationThetaOffsetUnits=deg  TranslationZOffset=0  TranslationZOffsetUnits=m
  Poussée et tenue à la main : Subsystem
  R du capteur : nesl_utility/PS-Simulink Converter  PhysicalDomain=network_engine_domain  SubClassName=ps_output  LeftPortType=input  RightPortType=output  PseudoPeriodic=off  Frequencies=[]  VectorFormat=inherit  Unit=1  AffineConversion=off
  Repère fixe (table) : sm_lib/Frames and Transforms/World Frame
  Retour aux axes du banc (roulis) : sm_lib/Frames and Transforms/Rigid Transform  RotationMethod=StandardAxis  FollAlignAxisA=+X  BaseAlignAxisA=+Y  FollAlignAxisB=+Y  BaseAlignAxisB=+Z  RotationStandardAxis=+Y  RotationAngle=-90  RotationAngleUnits=deg  RotationArbitraryAxis=[0 0 1]  RotationSequenceAxes=FollowerAxes  RotationSequence=XYX  RotationSequenceAngles=[0 0 0]  RotationSequenceAnglesUnits=deg  RotationMatrix=[1 0 0;0 1 0;0 0 1]  Quaternion=[1 0 0 0]  TranslationMethod=None  TranslationCartesianOffset=[0 0 0]  TranslationCartesianOffsetUnits=m  TranslationStandardAxis=+Z  TranslationStandardOffset=0  TranslationStandardOffsetUnits=m  TranslationROffset=0  TranslationROffsetUnits=m  TranslationThetaOffset=0  TranslationThetaOffsetUnits=deg  TranslationZOffset=0  TranslationZOffsetUnits=m
  Retour aux axes du banc (tangage) : sm_lib/Frames and Transforms/Rigid Transform  RotationMethod=StandardAxis  FollAlignAxisA=+X  BaseAlignAxisA=+Y  FollAlignAxisB=+Y  BaseAlignAxisB=+Z  RotationStandardAxis=+X  RotationAngle=90  RotationAngleUnits=deg  RotationArbitraryAxis=[0 0 1]  RotationSequenceAxes=FollowerAxes  RotationSequence=XYX  RotationSequenceAngles=[0 0 0]  RotationSequenceAnglesUnits=deg  RotationMatrix=[1 0 0;0 1 0;0 0 1]  Quaternion=[1 0 0 0]  TranslationMethod=None  TranslationCartesianOffset=[0 0 0]  TranslationCartesianOffsetUnits=m  TranslationStandardAxis=+Z  TranslationStandardOffset=0  TranslationStandardOffsetUnits=m  TranslationROffset=0  TranslationROffsetUnits=m  TranslationThetaOffset=0  TranslationThetaOffsetUnits=deg  TranslationZOffset=0  TranslationZOffsetUnits=m
  Roulis : sm_lib/Joints/Revolute Joint  Description=Pivot de roulis : 2 roulements 625, butées à ±butee_deg (goupille dans une lumière en arc), frottement b_cardan, raideur des câbles k_cables. Entrée mode : blocage_roulis (0 libre, 1 bloqué par la goupille).  JointMode=ProvidedByInput  CompositeWrenchDir=FollowerOnBase  CompositeWrenchFrame=BaseFrame  SenseConstraintForce=off  SenseConstraintTorque=off  SenseTotalForce=off  SenseTotalTorque=off  PositionTargetSpecify=on  PositionTargetPriority=High  PositionTargetValue=q0_deg(1)  PositionTargetValueUnits=deg  VelocityTargetSpecify=on  VelocityTargetPriority=High  VelocityTargetValue=0  VelocityTargetValueUnits=deg/s  EquilibriumPosition=0  EquilibriumPositionUnits=deg  SpringStiffness=k_cables  SpringStiffnessUnits=N*m/rad  DampingCoefficient=b_cardan  DampingCoefficientUnits=N*m*s/rad  LowerLimitSpecify=on  LowerLimitBound=-butee_deg  LowerLimitBoundUnits=deg  LowerLimitStiffness=k_butee  LowerLimitStiffnessUnits=N*m/rad  LowerLimitDamping=c_butee  LowerLimitDampingUnits=N*m*s/rad  LowerLimitTransitionRegionWidth=0.1  LowerLimitTransitionRegionWidthUnits=deg  UpperLimitSpecify=on  UpperLimitBound=butee_deg  UpperLimitBoundUnits=deg  UpperLimitStiffness=k_butee  UpperLimitStiffnessUnits=N*m/rad  UpperLimitDamping=c_butee  UpperLimitDampingUnits=N*m*s/rad  UpperLimitTransitionRegionWidth=0.1  UpperLimitTransitionRegionWidthUnits=deg  TorqueActuationMode=InputTorque  MotionActuationMode=ComputedMotion  SensePosition=on  SenseVelocity=on  SenseAcceleration=off  SenseTorqueForce=off  SenseLowerLimitTorqueForce=off  SenseUpperLimitTorqueForce=off
  Solveur Simscape : nesl_utility/Solver Configuration  PhysicalDomain=network_engine_domain  SubClassName=solver  LeftPortType=input  RightPortType=generic  Tones=[]  Harmonics=[]  SimulateNoise=off  Profile=off  UseLocalSampling=off  EnableSwitchedLinearOptims=on  FrequencyDomain=off  UseCCode=off  RelTol=0.001  AbsTol=0.001  MinStep=1e-09  ToWorkspace=off  RevertToSquareIcSolve=off  NumHomotopyIterations=100  PhasorMode=off  PhasorModeNumHarmonics=1  ConsistencySolver=NEWTON_XTOL_AFTER_FTOL  IndexReductionMethod=DerivativeReplacement  DoDC=off  ResidualTolerance=1e-09  ConsistencyTolSource=GLOBAL  ConsistencyAbsTol=0.001  ConsistencyRelTol=0.001  ConsistencyTolFactor=0.001  UseLocalSolver=off  LocalSolverChoice=NE_BACKWARD_EULER_ADVANCER  ResolveIndetEquations=on  FunctionEvalNumThread=1  LocalSolverSampleTime=0.001  DoFixedCost=off  MaxNonlinIter=3  MaxModeIter=2  ComputeImpulses=off  ImpulseIterations=2  LinearAlgebra=auto  LinearAlgebraNumThread=0  EquationFormulation=NE_TIME_EF  DelaysMemoryBudget=1024  AutomaticFiltering=on  FilteringTimeConstant=0.001  PartitionStorageMethod=AS_NEEDED  PartitionMemoryBudget=1024  PartitionMethod=ROBUST  MultibodyUseLocalSolver=off  MultibodyLocalSolverChoice=ODE1  MultibodyLocalSolverSampleTime=0.001
  Tangage : sm_lib/Joints/Revolute Joint  Description=Pivot de tangage : 2 roulements 625, butées à ±butee_deg (goupille dans une lumière en arc), frottement b_cardan, raideur des câbles k_cables. Entrée mode : blocage_tangage (0 libre, 1 bloqué par la goupille).  JointMode=ProvidedByInput  CompositeWrenchDir=FollowerOnBase  CompositeWrenchFrame=BaseFrame  SenseConstraintForce=off  SenseConstraintTorque=off  SenseTotalForce=off  SenseTotalTorque=off  PositionTargetSpecify=on  PositionTargetPriority=High  PositionTargetValue=q0_deg(2)  PositionTargetValueUnits=deg  VelocityTargetSpecify=on  VelocityTargetPriority=High  VelocityTargetValue=0  VelocityTargetValueUnits=deg/s  EquilibriumPosition=0  EquilibriumPositionUnits=deg  SpringStiffness=k_cables  SpringStiffnessUnits=N*m/rad  DampingCoefficient=b_cardan  DampingCoefficientUnits=N*m*s/rad  LowerLimitSpecify=on  LowerLimitBound=-butee_deg  LowerLimitBoundUnits=deg  LowerLimitStiffness=k_butee  LowerLimitStiffnessUnits=N*m/rad  LowerLimitDamping=c_butee  LowerLimitDampingUnits=N*m*s/rad  LowerLimitTransitionRegionWidth=0.1  LowerLimitTransitionRegionWidthUnits=deg  UpperLimitSpecify=on  UpperLimitBound=butee_deg  UpperLimitBoundUnits=deg  UpperLimitStiffness=k_butee  UpperLimitStiffnessUnits=N*m/rad  UpperLimitDamping=c_butee  UpperLimitDampingUnits=N*m*s/rad  UpperLimitTransitionRegionWidth=0.1  UpperLimitTransitionRegionWidthUnits=deg  TorqueActuationMode=InputTorque  MotionActuationMode=ComputedMotion  SensePosition=on  SenseVelocity=on  SenseAcceleration=off  SenseTorqueForce=off  SenseLowerLimitTorqueForce=off  SenseUpperLimitTorqueForce=off
  a du capteur : nesl_utility/PS-Simulink Converter  PhysicalDomain=network_engine_domain  SubClassName=ps_output  LeftPortType=input  RightPortType=output  PseudoPeriodic=off  Frequencies=[]  VectorFormat=inherit  Unit=m/s^2  AffineConversion=off
  angle roulis : nesl_utility/PS-Simulink Converter  PhysicalDomain=network_engine_domain  SubClassName=ps_output  LeftPortType=input  RightPortType=output  PseudoPeriodic=off  Frequencies=[]  VectorFormat=inherit  Unit=deg  AffineConversion=off
  angle tangage : nesl_utility/PS-Simulink Converter  PhysicalDomain=network_engine_domain  SubClassName=ps_output  LeftPortType=input  RightPortType=output  PseudoPeriodic=off  Frequencies=[]  VectorFormat=inherit  Unit=deg  AffineConversion=off
  couple roulis : nesl_utility/Simulink-PS Converter  PhysicalDomain=network_engine_domain  SubClassName=ps_input  LeftPortType=input  RightPortType=output  PseudoPeriodic=off  Frequencies=[]  NoiseDistribution=none  NoiseParameters=[]  Unit=N*m  AffineConversion=off  FilteringAndDerivatives=provide  SimscapeFilterOrder=1  InputFilterTimeConstant=0.001  UdotUserProvided=0
  couple tangage : nesl_utility/Simulink-PS Converter  PhysicalDomain=network_engine_domain  SubClassName=ps_input  LeftPortType=input  RightPortType=output  PseudoPeriodic=off  Frequencies=[]  NoiseDistribution=none  NoiseParameters=[]  Unit=N*m  AffineConversion=off  FilteringAndDerivatives=provide  SimscapeFilterOrder=1  InputFilterTimeConstant=0.001  UdotUserProvided=0
  mode roulis : nesl_utility/Simulink-PS Converter  PhysicalDomain=network_engine_domain  SubClassName=ps_input  LeftPortType=input  RightPortType=output  PseudoPeriodic=off  Frequencies=[]  NoiseDistribution=none  NoiseParameters=[]  Unit=1  AffineConversion=off  FilteringAndDerivatives=provide  SimscapeFilterOrder=1  InputFilterTimeConstant=0.001  UdotUserProvided=0
  mode tangage : nesl_utility/Simulink-PS Converter  PhysicalDomain=network_engine_domain  SubClassName=ps_input  LeftPortType=input  RightPortType=output  PseudoPeriodic=off  Frequencies=[]  NoiseDistribution=none  NoiseParameters=[]  Unit=1  AffineConversion=off  FilteringAndDerivatives=provide  SimscapeFilterOrder=1  InputFilterTimeConstant=0.001  UdotUserProvided=0
  omega {1..4} (4 alike) : nesl_utility/PS-Simulink Converter  PhysicalDomain=network_engine_domain  SubClassName=ps_output  LeftPortType=input  RightPortType=output  PseudoPeriodic=off  Frequencies=[]  VectorFormat=inherit  Unit=rad/s  AffineConversion=off
  omega du capteur : nesl_utility/PS-Simulink Converter  PhysicalDomain=network_engine_domain  SubClassName=ps_output  LeftPortType=input  RightPortType=output  PseudoPeriodic=off  Frequencies=[]  VectorFormat=inherit  Unit=rad/s  AffineConversion=off
  theta {1..4} (4 alike) : nesl_utility/PS-Simulink Converter  PhysicalDomain=network_engine_domain  SubClassName=ps_output  LeftPortType=input  RightPortType=output  PseudoPeriodic=off  Frequencies=[]  VectorFormat=inherit  Unit=rad  AffineConversion=off
  vitesse roulis : nesl_utility/PS-Simulink Converter  PhysicalDomain=network_engine_domain  SubClassName=ps_output  LeftPortType=input  RightPortType=output  PseudoPeriodic=off  Frequencies=[]  VectorFormat=inherit  Unit=deg/s  AffineConversion=off
  vitesse tangage : nesl_utility/PS-Simulink Converter  PhysicalDomain=network_engine_domain  SubClassName=ps_output  LeftPortType=input  RightPortType=output  PseudoPeriodic=off  Frequencies=[]  VectorFormat=inherit  Unit=deg/s  AffineConversion=off
  omega roues (rad par s) : Outport
  angles cardan (°) : Outport  Port=2
  vitesses cardan (° par s) : Outport  Port=3
  R capteur : Outport  Port=4
  omega capteur (rad par s) : Outport  Port=5
  a capteur (m par s²) : Outport  Port=6
  angle des roues (rad) : Outport  Port=7
  wires:
  Goupille roulis/1 -> mode roulis/1
  Goupille tangage/1 -> mode tangage/1
  Cm (N.m)/1 -> Demux Cm/1
  Demux Cm/1 -> Cm 1/1
  omega 1/1 -> Mux omega/1
  theta 1/1 -> Mux theta/1
  Demux Cm/2 -> Cm 2/1
  omega 2/1 -> Mux omega/2
  theta 2/1 -> Mux theta/2
  Demux Cm/3 -> Cm 3/1
  omega 3/1 -> Mux omega/3
  theta 3/1 -> Mux theta/3
  Demux Cm/4 -> Cm 4/1
  omega 4/1 -> Mux omega/4
  theta 4/1 -> Mux theta/4
  Mux omega/1 -> omega roues (rad par s)/1
  angle roulis/1 -> Mux angles/1
  vitesse roulis/1 -> Mux vitesses/1
  angle tangage/1 -> Mux angles/2
  vitesse tangage/1 -> Mux vitesses/2
  Mux angles/1 -> angles cardan (°)/1, [angles_deg]  "angles_deg"
  Mux vitesses/1 -> vitesses cardan (° par s)/1, [vitesses_dps]  "vitesses_dps"
  R du capteur/1 -> R capteur/1
  omega du capteur/1 -> omega capteur (rad par s)/1
  a du capteur/1 -> a capteur (m par s²)/1
  Mux theta/1 -> angle des roues (rad)/1
  [angles_deg] -> Poussée et tenue à la main/1(angles du cardan (°))
  [vitesses_dps] -> Poussée et tenue à la main/2(vitesses du cardan (° par s))
  Poussée et tenue à la main/1(couple sur les axes (N.m)) -> Axes du couple extérieur/1
  Axes du couple extérieur/1 -> [c_roulis]  "c_roulis"
  Axes du couple extérieur/2 -> [c_tangage]  "c_tangage"
  [c_roulis] -> couple roulis/1
  [c_tangage] -> couple tangage/1
  poussée (N.m)/1 -> Poussée et tenue à la main/3(poussée (N.m))
  connections:
  Pesanteur/RConn1 -- Solveur Simscape/RConn1 -- "Axe de roulis (X), au pivot"/LConn1 -- Repère fixe (table)/RConn1 -- "Bâti fixe (socle, poteau, fourche)"/LConn1 -- Mouvement du BNO055/LConn1
  mode roulis/RConn1 -- Roulis/LConn3
  "Axe de roulis (X), au pivot"/RConn1 -- Roulis/LConn1
  Roulis/RConn1 -- Retour aux axes du banc (roulis)/LConn1
  Croisillon (tourne en roulis)/LConn1 -- Retour aux axes du banc (roulis)/RConn1 -- Axe de tangage (Y)/LConn1
  mode tangage/RConn1 -- Tangage/LConn3
  Axe de tangage (Y)/RConn1 -- Tangage/LConn1
  Tangage/RConn1 -- Retour aux axes du banc (tangage)/LConn1
  Paliers de tangage/LConn1 -- Retour aux axes du banc (tangage)/RConn1 -- Position du pivot sur le corps/LConn1
  "Dispositif (corps, étage, électronique, câblage)"/LConn1 -- Position du pivot sur le corps/RConn1 -- Module de roue 3 (225°)/LConn1 -- Module de roue 4 (315°)/LConn1 -- Module de roue 2 (135°)/LConn1 -- Module de roue 1 (45°)/LConn1 -- Position du BNO055/LConn1
  Cm 1/RConn1 -- Module de roue 1 (45°)/LConn2
  Module de roue 1 (45°)/RConn1 -- omega 1/LConn1
  Module de roue 1 (45°)/RConn2 -- theta 1/LConn1
  Cm 2/RConn1 -- Module de roue 2 (135°)/LConn2
  Module de roue 2 (135°)/RConn1 -- omega 2/LConn1
  Module de roue 2 (135°)/RConn2 -- theta 2/LConn1
  Cm 3/RConn1 -- Module de roue 3 (225°)/LConn2
  Module de roue 3 (225°)/RConn1 -- omega 3/LConn1
  Module de roue 3 (225°)/RConn2 -- theta 3/LConn1
  Cm 4/RConn1 -- Module de roue 4 (315°)/LConn2
  Module de roue 4 (315°)/RConn1 -- omega 4/LConn1
  Module de roue 4 (315°)/RConn2 -- theta 4/LConn1
  Roulis/RConn2 -- angle roulis/LConn1
  Roulis/RConn3 -- vitesse roulis/LConn1
  Tangage/RConn2 -- angle tangage/LConn1
  Tangage/RConn3 -- vitesse tangage/LConn1
  Position du BNO055/RConn1 -- Mouvement du BNO055/RConn1
  Mouvement du BNO055/RConn2 -- R du capteur/LConn1
  Mouvement du BNO055/RConn3 -- omega du capteur/LConn1
  Mouvement du BNO055/RConn4 -- a du capteur/LConn1
  couple roulis/RConn1 -- Roulis/LConn2
  couple tangage/RConn1 -- Tangage/LConn2

== system jumeau_banc_rw/Procédé/Jumeau Simscape/Mécanique (CAO version 3)/Bâti fixe (socle, poteau, fourche) ==
  Fourche : sm_lib/Body Elements/File Solid  Description=|  ExtGeomFileName=RW-07_Fourche.stl  UnitType=Custom  ExtGeomFileUnits=mm  StepReaderType=HEX  ExportConvexHullGeometry=off  InertiaType=Custom  BasedOnType=DensityFromFile  Density=1000  DensityUnits=kg/m^3  Mass=0.029504459  MassUnits=kg  CenterOfMass=[-0.0003309437 -5.5717397e-19 -0.021775446]  CenterOfMassUnits=m  MomentsOfInertia=[7.9224425e-06 1.2711368e-05 9.6343008e-06]  MomentsOfInertiaUnits=kg*m^2  ProductsOfInertia=[2.3391402e-22 -9.9835768e-08 1.4118251e-22]  ProductsOfInertiaUnits=kg*m^2  GraphicType=FromGeometry  MarkerShape=Sphere  MarkerSize=10  GraphicVisPropType=SimpleVisualProperties  GraphicDiffuseColor=[0.576 0.471 0.376]  GraphicOpacity=1  GraphicSpecularColor=[0.5 0.5 0.5 1.0]  GraphicAmbientColor=[0.15 0.15 0.15 1.0]  GraphicEmissiveColor=[0.0 0.0 0.0 1.0]  GraphicShininess=75  DoExposeReferenceFrame=on  SerializedFrames=<Frames/>
      | Pièce CAO : Fourche (RW-07_Fourche)
      | Masse 29.50 g : PLA imprimé, 2 parois et 15 % de remplissage (hypothèse de conception), 800 kg/m³.
      | Centre de masse et inertie : calculés sur la géométrie de la CAO.
  Pose Fourche : sm_lib/Frames and Transforms/Rigid Transform  RotationMethod=None  FollAlignAxisA=+X  BaseAlignAxisA=+Y  FollAlignAxisB=+Y  BaseAlignAxisB=+Z  RotationStandardAxis=+Z  RotationAngle=0  RotationAngleUnits=deg  RotationArbitraryAxis=[0 0 1]  RotationSequenceAxes=FollowerAxes  RotationSequence=XYX  RotationSequenceAngles=[0 0 0]  RotationSequenceAnglesUnits=deg  RotationMatrix=[1 0 0;0 1 0;0 0 1]  Quaternion=[1 0 0 0]  TranslationMethod=Cartesian  TranslationCartesianOffset=[0 0 24]  TranslationCartesianOffsetUnits=mm  TranslationStandardAxis=+Z  TranslationStandardOffset=0  TranslationStandardOffsetUnits=m  TranslationROffset=0  TranslationROffsetUnits=m  TranslationThetaOffset=0  TranslationThetaOffsetUnits=deg  TranslationZOffset=0  TranslationZOffsetUnits=m
  Pose Poteau : sm_lib/Frames and Transforms/Rigid Transform  RotationMethod=None  FollAlignAxisA=+X  BaseAlignAxisA=+Y  FollAlignAxisB=+Y  BaseAlignAxisB=+Z  RotationStandardAxis=+Z  RotationAngle=0  RotationAngleUnits=deg  RotationArbitraryAxis=[0 0 1]  RotationSequenceAxes=FollowerAxes  RotationSequence=XYX  RotationSequenceAngles=[0 0 0]  RotationSequenceAnglesUnits=deg  RotationMatrix=[1 0 0;0 1 0;0 0 1]  Quaternion=[1 0 0 0]  TranslationMethod=Cartesian  TranslationCartesianOffset=[0 0 -134]  TranslationCartesianOffsetUnits=mm  TranslationStandardAxis=+Z  TranslationStandardOffset=0  TranslationStandardOffsetUnits=m  TranslationROffset=0  TranslationROffsetUnits=m  TranslationThetaOffset=0  TranslationThetaOffsetUnits=deg  TranslationZOffset=0  TranslationZOffsetUnits=m
  Pose Roulement de roulis 1 : sm_lib/Frames and Transforms/Rigid Transform  RotationMethod=RotationMatrix  FollAlignAxisA=+X  BaseAlignAxisA=+Y  FollAlignAxisB=+Y  BaseAlignAxisB=+Z  RotationStandardAxis=+Z  RotationAngle=0  RotationAngleUnits=deg  RotationArbitraryAxis=[0 0 1]  RotationSequenceAxes=FollowerAxes  RotationSequence=XYX  RotationSequenceAngles=[0 0 0]  RotationSequenceAnglesUnits=deg  RotationMatrix=[0 0 1;1 0 0;0 1 0]  Quaternion=[1 0 0 0]  TranslationMethod=Cartesian  TranslationCartesianOffset=[18 0 24]  TranslationCartesianOffsetUnits=mm  TranslationStandardAxis=+Z  TranslationStandardOffset=0  TranslationStandardOffsetUnits=m  TranslationROffset=0  TranslationROffsetUnits=m  TranslationThetaOffset=0  TranslationThetaOffsetUnits=deg  TranslationZOffset=0  TranslationZOffsetUnits=m
  Pose Roulement de roulis 2 : sm_lib/Frames and Transforms/Rigid Transform  RotationMethod=RotationMatrix  FollAlignAxisA=+X  BaseAlignAxisA=+Y  FollAlignAxisB=+Y  BaseAlignAxisB=+Z  RotationStandardAxis=+Z  RotationAngle=0  RotationAngleUnits=deg  RotationArbitraryAxis=[0 0 1]  RotationSequenceAxes=FollowerAxes  RotationSequence=XYX  RotationSequenceAngles=[0 0 0]  RotationSequenceAnglesUnits=deg  RotationMatrix=[0 0 -1;1 0 0;0 -1 0]  Quaternion=[1 0 0 0]  TranslationMethod=Cartesian  TranslationCartesianOffset=[-18 0 24]  TranslationCartesianOffsetUnits=mm  TranslationStandardAxis=+Z  TranslationStandardOffset=0  TranslationStandardOffsetUnits=m  TranslationROffset=0  TranslationROffsetUnits=m  TranslationThetaOffset=0  TranslationThetaOffsetUnits=deg  TranslationZOffset=0  TranslationZOffsetUnits=m
  Pose Socle : sm_lib/Frames and Transforms/Rigid Transform  RotationMethod=None  FollAlignAxisA=+X  BaseAlignAxisA=+Y  FollAlignAxisB=+Y  BaseAlignAxisB=+Z  RotationStandardAxis=+Z  RotationAngle=0  RotationAngleUnits=deg  RotationArbitraryAxis=[0 0 1]  RotationSequenceAxes=FollowerAxes  RotationSequence=XYX  RotationSequenceAngles=[0 0 0]  RotationSequenceAnglesUnits=deg  RotationMatrix=[1 0 0;0 1 0;0 0 1]  Quaternion=[1 0 0 0]  TranslationMethod=Cartesian  TranslationCartesianOffset=[0 0 -132]  TranslationCartesianOffsetUnits=mm  TranslationStandardAxis=+Z  TranslationStandardOffset=0  TranslationStandardOffsetUnits=m  TranslationROffset=0  TranslationROffsetUnits=m  TranslationThetaOffset=0  TranslationThetaOffsetUnits=deg  TranslationZOffset=0  TranslationZOffsetUnits=m
  Poteau : sm_lib/Body Elements/File Solid  Description=|  ExtGeomFileName=RW-25_Tube-12x1.stl  UnitType=Custom  ExtGeomFileUnits=mm  StepReaderType=HEX  ExportConvexHullGeometry=off  InertiaType=Custom  BasedOnType=DensityFromFile  Density=1000  DensityUnits=kg/m^3  Mass=0.012689521  MassUnits=kg  CenterOfMass=[-2.3222018e-18 -2.1647994e-19 0.068]  CenterOfMassUnits=m  MomentsOfInertia=[1.9752297e-05 1.9752297e-05 3.8703039e-07]  MomentsOfInertiaUnits=kg*m^2  ProductsOfInertia=[-3.0481738e-23 -7.4651325e-22 2.3489905e-23]  ProductsOfInertiaUnits=kg*m^2  GraphicType=FromGeometry  MarkerShape=Sphere  MarkerSize=10  GraphicVisPropType=SimpleVisualProperties  GraphicDiffuseColor=[0.6 0.6 0.6]  GraphicOpacity=1  GraphicSpecularColor=[0.5 0.5 0.5 1.0]  GraphicAmbientColor=[0.15 0.15 0.15 1.0]  GraphicEmissiveColor=[0.0 0.0 0.0 1.0]  GraphicShininess=75  DoExposeReferenceFrame=on  SerializedFrames=<Frames/>
      | Pièce CAO : Poteau (RW-25_Tube-12x1)
      | Masse 12.69 g : aluminium, 2700 kg/m³.
      | Centre de masse et inertie : calculés sur la géométrie de la CAO.
  Roulement de roulis 1 : sm_lib/Body Elements/File Solid  Description=|  ExtGeomFileName=RW-20_Roulement-625.stl  UnitType=Custom  ExtGeomFileUnits=mm  StepReaderType=HEX  ExportConvexHullGeometry=off  InertiaType=Custom  BasedOnType=DensityFromFile  Density=1000  DensityUnits=kg/m^3  Mass=0.0044  MassUnits=kg  CenterOfMass=[-4.3080529e-19 -4.0130534e-19 0.0025]  CenterOfMassUnits=m  MomentsOfInertia=[8.6441667e-08 8.6441667e-08 1.5455e-07]  MomentsOfInertiaUnits=kg*m^2  ProductsOfInertia=[-6.0797928e-26 -7.409851e-25 8.4651334e-24]  ProductsOfInertiaUnits=kg*m^2  GraphicType=FromGeometry  MarkerShape=Sphere  MarkerSize=10  GraphicVisPropType=SimpleVisualProperties  GraphicDiffuseColor=[0.627 0.627 0.627]  GraphicOpacity=1  GraphicSpecularColor=[0.5 0.5 0.5 1.0]  GraphicAmbientColor=[0.15 0.15 0.15 1.0]  GraphicEmissiveColor=[0.0 0.0 0.0 1.0]  GraphicShininess=75  DoExposeReferenceFrame=on  SerializedFrames=<Frames/>
      | Pièce CAO : Roulement de roulis 1 (RW-20_Roulement-625)
      | Masse 4.40 g : roulement 625, catalogue, 4,4 g répartis sur le volume de la CAO.
      | Centre de masse et inertie : calculés sur la géométrie de la CAO.
  Roulement de roulis 2 : sm_lib/Body Elements/File Solid  Description=|  ExtGeomFileName=RW-20_Roulement-625.stl  UnitType=Custom  ExtGeomFileUnits=mm  StepReaderType=HEX  ExportConvexHullGeometry=off  InertiaType=Custom  BasedOnType=DensityFromFile  Density=1000  DensityUnits=kg/m^3  Mass=0.0044  MassUnits=kg  CenterOfMass=[-4.3080529e-19 -4.0130534e-19 0.0025]  CenterOfMassUnits=m  MomentsOfInertia=[8.6441667e-08 8.6441667e-08 1.5455e-07]  MomentsOfInertiaUnits=kg*m^2  ProductsOfInertia=[-6.0797928e-26 -7.409851e-25 8.4651334e-24]  ProductsOfInertiaUnits=kg*m^2  GraphicType=FromGeometry  MarkerShape=Sphere  MarkerSize=10  GraphicVisPropType=SimpleVisualProperties  GraphicDiffuseColor=[0.627 0.627 0.627]  GraphicOpacity=1  GraphicSpecularColor=[0.5 0.5 0.5 1.0]  GraphicAmbientColor=[0.15 0.15 0.15 1.0]  GraphicEmissiveColor=[0.0 0.0 0.0 1.0]  GraphicShininess=75  DoExposeReferenceFrame=on  SerializedFrames=<Frames/>
      | Pièce CAO : Roulement de roulis 2 (RW-20_Roulement-625)
      | Masse 4.40 g : roulement 625, catalogue, 4,4 g répartis sur le volume de la CAO.
      | Centre de masse et inertie : calculés sur la géométrie de la CAO.
  Socle : sm_lib/Body Elements/File Solid  Description=|  ExtGeomFileName=RW-10_Socle.stl  UnitType=Custom  ExtGeomFileUnits=mm  StepReaderType=HEX  ExportConvexHullGeometry=off  InertiaType=Custom  BasedOnType=DensityFromFile  Density=1000  DensityUnits=kg/m^3  Mass=0.33790201  MassUnits=kg  CenterOfMass=[-5.2014279e-05 -2.6326472e-17 0.00099137492]  CenterOfMassUnits=m  MomentsOfInertia=[0.0013974228 0.0013972208 0.0027224801]  MomentsOfInertiaUnits=kg*m^2  ProductsOfInertia=[1.4388294e-19 4.7291186e-07 8.5112653e-20]  ProductsOfInertiaUnits=kg*m^2  GraphicType=FromGeometry  MarkerShape=Sphere  MarkerSize=10  GraphicVisPropType=SimpleVisualProperties  GraphicDiffuseColor=[0.576 0.471 0.376]  GraphicOpacity=1  GraphicSpecularColor=[0.5 0.5 0.5 1.0]  GraphicAmbientColor=[0.15 0.15 0.15 1.0]  GraphicEmissiveColor=[0.0 0.0 0.0 1.0]  GraphicShininess=75  DoExposeReferenceFrame=on  SerializedFrames=<Frames/>
      | Pièce CAO : Socle (RW-10_Socle)
      | Masse 337.90 g : PLA imprimé, 2 parois et 15 % de remplissage (hypothèse de conception), 800 kg/m³.
      | Centre de masse et inertie : calculés sur la géométrie de la CAO.
  F : PMIOPort  Side=Left
  connections:
  Pose Socle/LConn1 -- F/RConn1 -- Pose Poteau/LConn1 -- Pose Fourche/LConn1 -- Pose Roulement de roulis 1/LConn1 -- Pose Roulement de roulis 2/LConn1
  Pose Socle/RConn1 -- Socle/RConn1
  Pose Poteau/RConn1 -- Poteau/RConn1
  Pose Fourche/RConn1 -- Fourche/RConn1
  Pose Roulement de roulis 1/RConn1 -- Roulement de roulis 1/RConn1
  Pose Roulement de roulis 2/RConn1 -- Roulement de roulis 2/RConn1
